simulink model "A_ZH_Z4"  (R2026a)
settings: Solver=VariableStepAuto  StopTime=20e-3  MaxStep=(185e-6)/25
settings Model: Creator=Szalay  LastModifiedBy=Szalay

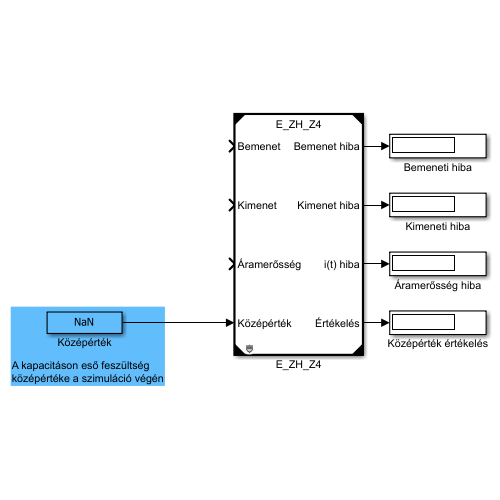
[thumbnail: Simulink's stored preview of the top-level diagram]
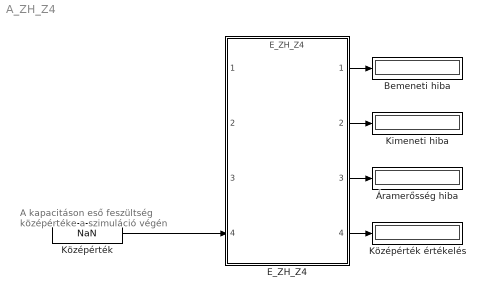
== system A_ZH_Z4 ==
  note: A kapacitáson eső feszültség
      | középértéke a szimuláció végén
  Bemeneti hiba : Display
  E_ZH_Z4 : ModelReference  ModelNameDialog=E_ZH_Z4.slxp  ModelReferenceVersion=3.5  CopyOfModelProtected=on
  Kimeneti hiba : Display
  Középérték : Constant  Value=NaN
  Középérték értékelés : Display
  Áramerősség hiba : Display
  wires:
  Középérték/1 -> E_ZH_Z4/4
  E_ZH_Z4/4 -> Középérték értékelés/1
  E_ZH_Z4/2 -> Kimeneti hiba/1
  E_ZH_Z4/1 -> Bemeneti hiba/1
  E_ZH_Z4/3 -> Áramerősség hiba/1
